simulink model "simrt_dio_loopback"  (R2024b)
settings: Solver=FixedStepDiscrete  StartTime=0.0  StopTime=inf  FixedStep=0.001  RelTol=1e-3
model workspace (MAT data in the model file):
  DIO_Automatic = Simulink.Parameter
  DIO_Automatic.Value = 0
  DIO_Automatic.Complexity = 'real'
  DIO_Automatic.Dimensions = [1 1]
  DIO_Automatic.Description = '1: one active output per second; 0: hold the manual bit mask.'
  DIO_Automatic.DataType = 'uint8'
  DIO_Automatic.Min = 0
  DIO_Automatic.Max = 1
  DIO_CheckLoopback = Simulink.Parameter
  DIO_CheckLoopback.Value = 0
  DIO_CheckLoopback.Complexity = 'real'
  DIO_CheckLoopback.Dimensions = [1 1]
  DIO_CheckLoopback.Description = 'Enable only with DIO0..3 wired to DIO4..7. Leave at 0 for meter tests.'
  DIO_CheckLoopback.DataType = 'uint8'
  DIO_CheckLoopback.Min = 0
  DIO_CheckLoopback.Max = 1
  DIO_Enable = Simulink.Parameter
  DIO_Enable.Value = 0
  DIO_Enable.Complexity = 'real'
  DIO_Enable.Dimensions = [1 1]
  DIO_Enable.Description = '0 drives all four outputs low; 1 enables the selected pattern.'
  DIO_Enable.DataType = 'uint8'
  DIO_Enable.Min = 0
  DIO_Enable.Max = 1
  DIO_ManualMask = Simulink.Parameter
  DIO_ManualMask.Value = 0
  DIO_ManualMask.Complexity = 'real'
  DIO_ManualMask.Dimensions = [1 1]
  DIO_ManualMask.Description = 'Bit 0..3 control DIO0..3 in manual mode.'
  DIO_ManualMask.DataType = 'uint8'
  DIO_ManualMask.Min = 0
  DIO_ManualMask.Max = 15
libraries: simrt_dio_library x4
settings Model: Creator=yonggang.zhang  LastModifiedBy=yonggang.zhang
settings OptimizationCC: EnhancedBackFolding=on  PassReuseOutputArgsAs=Individual arguments  ZeroExternalMemoryAtStartup=off  ZeroInternalMemoryAtStartup=off  MaxStackSize=64  OptimizeBlockOrder=speed  DifferentSizesBufferReuse=on  OptimizationCustomize=off  EfficientTunableParamExpr=on
settings DebuggingCC: ParameterTunabilityLossMsg=error
settings HardwareCC: ProdBitPerLong=64  ProdHWDeviceType=Intel->x86-64 (Linux 64)
settings SFSimCC: MATLABDynamicMemAlloc=off
settings RTWCC: Description=Embedded Coder  SystemTargetFile=ert.tlc  HardwareBoard=SimRT  TLCOptions="-aInlineSetEventsForThisBaseRateFcn=TLC_FALSE -aSuppressMultiTaskScheduler=TLC_FALSE  -aRateBasedStepFcn=0"  TemplateMakefile=ert_default_tmf  Toolchain=SimRT portable-linux-toolchain
settings CodeAppCC: ForceParamTrailComments=on  IgnoreCustomStorageClasses=off  OperatorAnnotations=on  SimulinkDataObjDesc=on  SFDataObjDesc=on  InsertBlockDesc=on
settings ERTTargetCC: ExtMode=on  ExtModeTransport=2  ExtModeStaticAlloc=on  ExtModeMexFile=ext_xcp  ExtModeIntrfLevel=Level2 - Open  InlinedParameterPlacement=Hierarchical

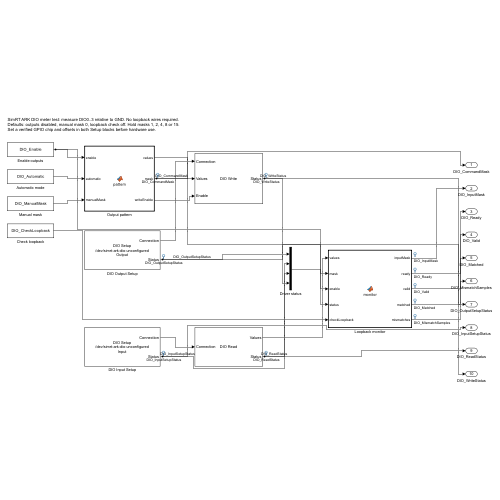
[thumbnail: Simulink's stored preview of the top-level diagram]
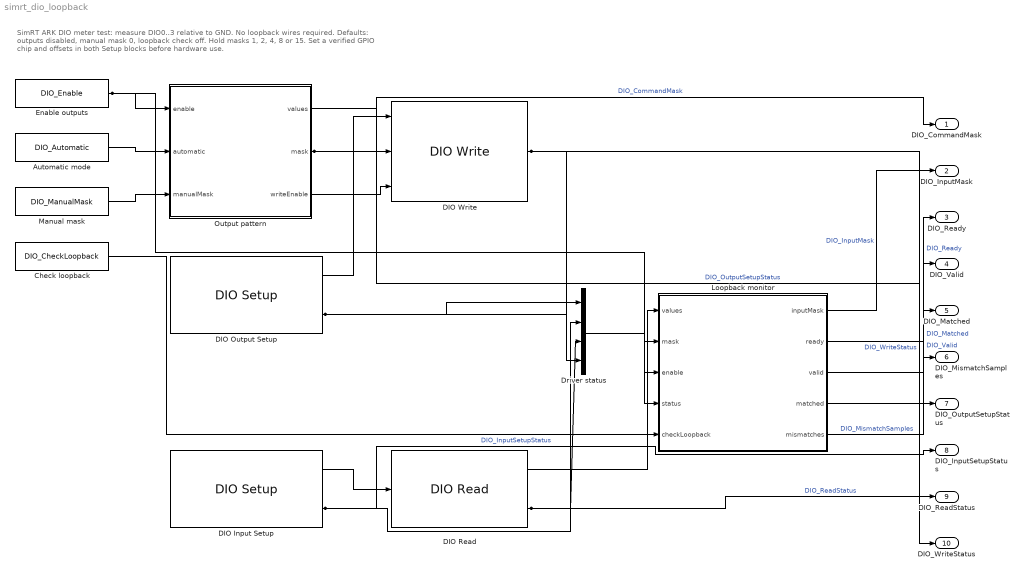
== system simrt_dio_loopback ==
  note: SimRT ARK DIO meter test: measure DIO0..3 relative to GND. No loopback wires required.
      | Defaults: outputs disabled, manual mask 0, loopback check off. Hold masks 1, 2, 4, 8 or 15.
      | Set a verified GPIO chip and offsets in both Setup blocks before hardware use.
  Automatic mode : Constant  Value=DIO_Automatic  SampleTime=0.001
  Check loopback : Constant  Value=DIO_CheckLoopback  SampleTime=0.001
  DIO Input Setup : simrt_dio_library/DIO Setup  Device=/dev/simrt-ark-dio-unconfigured  LineOffsets=[4 5 6 7]  Direction=Input  ActiveLow=false  InitialValues=false  SampleTime=0.001
  DIO Output Setup : simrt_dio_library/DIO Setup  Device=/dev/simrt-ark-dio-unconfigured  LineOffsets=[0 1 2 3]  Direction=Output  ActiveLow=false  InitialValues=false  SampleTime=0.001
  DIO Read : simrt_dio_library/DIO Read  LineCount=4
  DIO Write : simrt_dio_library/DIO Write
  Driver status : Mux
  Enable outputs : Constant  Value=DIO_Enable  SampleTime=0.001
  Loopback monitor : MATLAB Function  TreatAsAtomicUnit=on
  Manual mask : Constant  Value=DIO_ManualMask  SampleTime=0.001
  Output pattern : MATLAB Function  TreatAsAtomicUnit=on
  DIO_CommandMask : Outport
  DIO_InputMask : Outport  Port=2
  DIO_Ready : Outport  Port=3
  DIO_Valid : Outport  Port=4
  DIO_Matched : Outport  Port=5
  DIO_MismatchSamples : Outport  Port=6
  DIO_OutputSetupStatus : Outport  Port=7
  DIO_InputSetupStatus : Outport  Port=8
  DIO_ReadStatus : Outport  Port=9
  DIO_WriteStatus : Outport  Port=10
  wires:
  Enable outputs/1 -> Output pattern/1(enable), Loopback monitor/3(enable)
  Automatic mode/1 -> Output pattern/2(automatic)
  Manual mask/1 -> Output pattern/3(manualMask)
  DIO Output Setup/1 -> DIO Write/1
  Output pattern/1(values) -> DIO Write/2
  Output pattern/3(writeEnable) -> DIO Write/3
  DIO Input Setup/1 -> DIO Read/1
  DIO Output Setup/2 -> Driver status/1, DIO_OutputSetupStatus/1  "DIO_OutputSetupStatus"
  DIO Input Setup/2 -> Driver status/2, DIO_InputSetupStatus/1  "DIO_InputSetupStatus"
  DIO Read/2 -> Driver status/3, DIO_ReadStatus/1  "DIO_ReadStatus"
  DIO Write/1 -> Driver status/4, DIO_WriteStatus/1  "DIO_WriteStatus"
  DIO Read/1 -> Loopback monitor/1(values)
  Output pattern/2(mask) -> Loopback monitor/2(mask), DIO_CommandMask/1  "DIO_CommandMask"
  Driver status/1 -> Loopback monitor/4(status)
  Check loopback/1 -> Loopback monitor/5(checkLoopback)
  Loopback monitor/1(inputMask) -> DIO_InputMask/1  "DIO_InputMask"
  Loopback monitor/2(ready) -> DIO_Ready/1  "DIO_Ready"
  Loopback monitor/3(valid) -> DIO_Valid/1  "DIO_Valid"
  Loopback monitor/4(matched) -> DIO_Matched/1  "DIO_Matched"
  Loopback monitor/5(mismatches) -> DIO_MismatchSamples/1  "DIO_MismatchSamples"

== matlab function simrt_dio_loopback/Loopback monitor ==
  data: values input; inputMask output; mask input; enable input; status input; checkLoopback input; ready output; valid output; matched output; mismatches output
function [inputMask, ready, valid, matched, mismatches] = monitor(values, mask, enable, status, checkLoopback)
[inputMask, ready, valid, matched, mismatches] = simrtlinux.dio.loopbackMonitor(values, mask, enable, status, checkLoopback);
end

== matlab function simrt_dio_loopback/Output pattern ==
  data: enable input; values output; automatic input; manualMask input; mask output; writeEnable output
function [values, mask, writeEnable] = pattern(enable, automatic, manualMask)
[values, mask] = simrtlinux.dio.loopbackPattern(enable, automatic, manualMask);
writeEnable = true;
end
